simulink model "SITRA_S5_Physical"  (R2026a)
settings: Solver=daessc  StopTime=S5.stopTime  MaxStep=S5.maxStep  RelTol=1e-6  AbsTol=1e-9
values from neighbouring files (symbols this model uses):
  S5 = default_signals(S5)    [build_SITRA_S5_Physical.m]    (also in run_controllers_on_S5_physical.m = evalin('base', 'S5'); test_SITRA_S5_Physical.m = evalin('base', 'S5'); upgrade_electrical_subsystems.m = [model '/05_Power_Electronics'])
libraries: fl_lib x39, nesl_utility x23, ee_lib x9, simulink x8, slpidlib x1
(part 2 of 2)

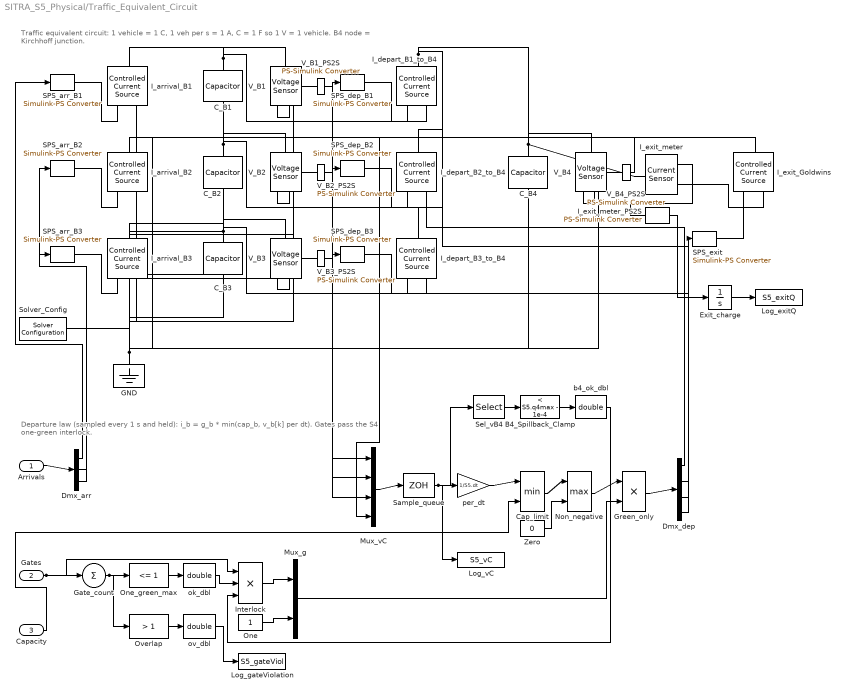
== system SITRA_S5_Physical/Traffic_Equivalent_Circuit ==
  note: Traffic equivalent circuit: 1 vehicle = 1 C, 1 veh per s = 1 A, C = 1 F so 1 V = 1 vehicle. B4 node = Kirchhoff junction.
  note: Departure law (sampled every 1 s and held): i_b = g_b * min(cap_b, v_b[k] per dt). Gates pass the S4 one-green interlock.
  Arrivals : Inport
  Gates : Inport  Port=2
  Capacity : Inport  Port=3
  B4_Spillback_Clamp : simulink/Logic and Bit Operations/Compare To Constant  relop=<  const=S5.q4max - 1e-4  OutDataTypeStr=boolean
  C_B1 : fl_lib/Electrical/Electrical Elements/Capacitor  c=S5.C_queue F  r=1e-6 Ohm  g=0 1/Ohm  i_specify=off  i_priority=None  i=0 A  i_nominal_specify=off  i_nominal_value=1  i_nominal_unit=A  v_specify=off  v_priority=None  v=0 V  v_nominal_specify=off  v_nominal_value=1  v_nominal_unit=V  vc_specify=on  vc_priority=High  vc=S5.vC0(1) V  vc_nominal_specify=off  vc_nominal_value=1  vc_nominal_unit=V
  C_B2 : fl_lib/Electrical/Electrical Elements/Capacitor  c=S5.C_queue F  r=1e-6 Ohm  g=0 1/Ohm  i_specify=off  i_priority=None  i=0 A  i_nominal_specify=off  i_nominal_value=1  i_nominal_unit=A  v_specify=off  v_priority=None  v=0 V  v_nominal_specify=off  v_nominal_value=1  v_nominal_unit=V  vc_specify=on  vc_priority=High  vc=S5.vC0(2) V  vc_nominal_specify=off  vc_nominal_value=1  vc_nominal_unit=V
  C_B3 : fl_lib/Electrical/Electrical Elements/Capacitor  c=S5.C_queue F  r=1e-6 Ohm  g=0 1/Ohm  i_specify=off  i_priority=None  i=0 A  i_nominal_specify=off  i_nominal_value=1  i_nominal_unit=A  v_specify=off  v_priority=None  v=0 V  v_nominal_specify=off  v_nominal_value=1  v_nominal_unit=V  vc_specify=on  vc_priority=High  vc=S5.vC0(3) V  vc_nominal_specify=off  vc_nominal_value=1  vc_nominal_unit=V
  C_B4 : fl_lib/Electrical/Electrical Elements/Capacitor  c=S5.C_queue F  r=1e-6 Ohm  g=0 1/Ohm  i_specify=off  i_priority=None  i=0 A  i_nominal_specify=off  i_nominal_value=1  i_nominal_unit=A  v_specify=off  v_priority=None  v=0 V  v_nominal_specify=off  v_nominal_value=1  v_nominal_unit=V  vc_specify=on  vc_priority=High  vc=S5.vC0(4) V  vc_nominal_specify=off  vc_nominal_value=1  vc_nominal_unit=V
  Cap_limit : MinMax  Inputs=2
  Dmx_arr : Demux  Outputs=3
  Dmx_dep : Demux
  Exit_charge : Integrator
  GND : fl_lib/Electrical/Electrical Elements/Electrical Reference
  Gate_count : Sum  Inputs=+
  Green_only : Product  Inputs=**
  I_arrival_B1 : fl_lib/Electrical/Electrical Sources/Controlled Current Source
  I_arrival_B2 : fl_lib/Electrical/Electrical Sources/Controlled Current Source
  I_arrival_B3 : fl_lib/Electrical/Electrical Sources/Controlled Current Source
  I_depart_B1_to_B4 : fl_lib/Electrical/Electrical Sources/Controlled Current Source
  I_depart_B2_to_B4 : fl_lib/Electrical/Electrical Sources/Controlled Current Source
  I_depart_B3_to_B4 : fl_lib/Electrical/Electrical Sources/Controlled Current Source
  I_exit_Goldwins : fl_lib/Electrical/Electrical Sources/Controlled Current Source
  I_exit_meter : fl_lib/Electrical/Electrical Sensors/Current Sensor
  I_exit_meter_PS2S : nesl_utility/PS-Simulink Converter  PhysicalDomain=network_engine_domain  SubClassName=ps_output  LeftPortType=input  RightPortType=output  PseudoPeriodic=off  Frequencies=[]  VectorFormat=inherit  Unit=A  AffineConversion=off
  Interlock : Product  Inputs=***
  Log_exitQ : ToWorkspace  VariableName=S5_exitQ  SaveFormat=Structure With Time  SampleTime=S5.dt
  Log_gateViolation : ToWorkspace  VariableName=S5_gateViol  SaveFormat=Structure With Time  SampleTime=1
  Log_vC : ToWorkspace  VariableName=S5_vC  SaveFormat=Structure With Time  SampleTime=S5.dt
  Mux_g : Mux  Inputs=2
  Mux_vC : Mux
  Non_negative : MinMax  Function=max  Inputs=2
  One : Constant
  One_green_max : simulink/Logic and Bit Operations/Compare To Constant  relop=<=  const=1  OutDataTypeStr=boolean
  Overlap : simulink/Logic and Bit Operations/Compare To Constant  relop=>  const=1  OutDataTypeStr=boolean
  SPS_arr_B1 : nesl_utility/Simulink-PS Converter  PhysicalDomain=network_engine_domain  SubClassName=ps_input  LeftPortType=input  RightPortType=output  PseudoPeriodic=off  Frequencies=[]  NoiseDistribution=none  NoiseParameters=[]  Unit=A  AffineConversion=off  FilteringAndDerivatives=zero  SimscapeFilterOrder=1  InputFilterTimeConstant=0.001  UdotUserProvided=0
  SPS_arr_B2 : nesl_utility/Simulink-PS Converter  PhysicalDomain=network_engine_domain  SubClassName=ps_input  LeftPortType=input  RightPortType=output  PseudoPeriodic=off  Frequencies=[]  NoiseDistribution=none  NoiseParameters=[]  Unit=A  AffineConversion=off  FilteringAndDerivatives=zero  SimscapeFilterOrder=1  InputFilterTimeConstant=0.001  UdotUserProvided=0
  SPS_arr_B3 : nesl_utility/Simulink-PS Converter  PhysicalDomain=network_engine_domain  SubClassName=ps_input  LeftPortType=input  RightPortType=output  PseudoPeriodic=off  Frequencies=[]  NoiseDistribution=none  NoiseParameters=[]  Unit=A  AffineConversion=off  FilteringAndDerivatives=zero  SimscapeFilterOrder=1  InputFilterTimeConstant=0.001  UdotUserProvided=0
  SPS_dep_B1 : nesl_utility/Simulink-PS Converter  PhysicalDomain=network_engine_domain  SubClassName=ps_input  LeftPortType=input  RightPortType=output  PseudoPeriodic=off  Frequencies=[]  NoiseDistribution=none  NoiseParameters=[]  Unit=A  AffineConversion=off  FilteringAndDerivatives=zero  SimscapeFilterOrder=1  InputFilterTimeConstant=0.001  UdotUserProvided=0
  SPS_dep_B2 : nesl_utility/Simulink-PS Converter  PhysicalDomain=network_engine_domain  SubClassName=ps_input  LeftPortType=input  RightPortType=output  PseudoPeriodic=off  Frequencies=[]  NoiseDistribution=none  NoiseParameters=[]  Unit=A  AffineConversion=off  FilteringAndDerivatives=zero  SimscapeFilterOrder=1  InputFilterTimeConstant=0.001  UdotUserProvided=0
  SPS_dep_B3 : nesl_utility/Simulink-PS Converter  PhysicalDomain=network_engine_domain  SubClassName=ps_input  LeftPortType=input  RightPortType=output  PseudoPeriodic=off  Frequencies=[]  NoiseDistribution=none  NoiseParameters=[]  Unit=A  AffineConversion=off  FilteringAndDerivatives=zero  SimscapeFilterOrder=1  InputFilterTimeConstant=0.001  UdotUserProvided=0
  SPS_exit : nesl_utility/Simulink-PS Converter  PhysicalDomain=network_engine_domain  SubClassName=ps_input  LeftPortType=input  RightPortType=output  PseudoPeriodic=off  Frequencies=[]  NoiseDistribution=none  NoiseParameters=[]  Unit=A  AffineConversion=off  FilteringAndDerivatives=zero  SimscapeFilterOrder=1  InputFilterTimeConstant=0.001  UdotUserProvided=0
  Sample_queue : ZeroOrderHold  SampleTime=S5.dt
  Sel_vB4 : Selector  InputPortWidth=4  IndexOptions=Index vector (dialog)  Indices=4  OutputSizes=1
  Solver_Config : nesl_utility/Solver Configuration  PhysicalDomain=network_engine_domain  SubClassName=solver  LeftPortType=input  RightPortType=generic  Tones=[]  Harmonics=[]  SimulateNoise=off  Profile=off  UseLocalSampling=off  EnableSwitchedLinearOptims=on  FrequencyDomain=off  UseCCode=off  RelTol=0.001  AbsTol=0.001  MinStep=1e-09  ToWorkspace=off  RevertToSquareIcSolve=off  NumHomotopyIterations=100  PhasorMode=off  PhasorModeNumHarmonics=1  ConsistencySolver=NEWTON_XTOL_AFTER_FTOL  CanonicalOrdering=CANONICAL  OptimizeIntermediates=OPTIMIZED  IndexReductionMethod=DerivativeReplacement  DoDC=off  ResidualTolerance=1e-09  ConsistencyTolSource=GLOBAL  ConsistencyAbsTol=0.001  ConsistencyRelTol=0.001  ConsistencyTolFactor=0.001  UseLocalSolver=off  LocalSolverChoice=NE_BACKWARD_EULER_ADVANCER  ResolveIndetEquations=on  FunctionEvalNumThread=1  LocalSolverSampleTime=0.001  DoFixedCost=off  MaxNonlinIter=3  MaxModeIter=2  ComputeImpulses=off  ImpulseIterations=2  LinearAlgebra=auto  LinearAlgebraNumThread=0  EquationFormulation=NE_TIME_EF  DelaysMemoryBudget=1024  AutomaticFiltering=on  FilteringTimeConstant=0.001  PartitionStorageMethod=AS_NEEDED  PartitionMemoryBudget=1024  PartitionMethod=ROBUST  MultibodyUseLocalSolver=off  MultibodyLocalSolverChoice=ODE1  MultibodyLocalSolverSampleTime=0.001
  V_B{1..4} (4 alike) : fl_lib/Electrical/Electrical Sensors/Voltage Sensor
  V_B1_PS2S : nesl_utility/PS-Simulink Converter  PhysicalDomain=network_engine_domain  SubClassName=ps_output  LeftPortType=input  RightPortType=output  PseudoPeriodic=off  Frequencies=[]  VectorFormat=inherit  Unit=V  AffineConversion=off
  V_B2_PS2S : nesl_utility/PS-Simulink Converter  PhysicalDomain=network_engine_domain  SubClassName=ps_output  LeftPortType=input  RightPortType=output  PseudoPeriodic=off  Frequencies=[]  VectorFormat=inherit  Unit=V  AffineConversion=off
  V_B3_PS2S : nesl_utility/PS-Simulink Converter  PhysicalDomain=network_engine_domain  SubClassName=ps_output  LeftPortType=input  RightPortType=output  PseudoPeriodic=off  Frequencies=[]  VectorFormat=inherit  Unit=V  AffineConversion=off
  V_B4_PS2S : nesl_utility/PS-Simulink Converter  PhysicalDomain=network_engine_domain  SubClassName=ps_output  LeftPortType=input  RightPortType=output  PseudoPeriodic=off  Frequencies=[]  VectorFormat=inherit  Unit=V  AffineConversion=off
  Zero : Constant  Value=0
  b4_ok_dbl : DataTypeConversion  OutDataTypeStr=double  SaturateOnIntegerOverflow=off  RndMeth=Floor
  ok_dbl : DataTypeConversion  OutDataTypeStr=double  SaturateOnIntegerOverflow=off  RndMeth=Floor
  ov_dbl : DataTypeConversion  OutDataTypeStr=double  SaturateOnIntegerOverflow=off  RndMeth=Floor
  per_dt : Gain  Gain=1/S5.dt
  wires:
  Arrivals/1 -> Dmx_arr/1
  Dmx_arr/1 -> SPS_arr_B1/1
  Dmx_arr/2 -> SPS_arr_B2/1
  Dmx_arr/3 -> SPS_arr_B3/1
  Gates/1 -> Gate_count/1, Interlock/1
  Gate_count/1 -> One_green_max/1, Overlap/1
  One_green_max/1 -> ok_dbl/1
  ok_dbl/1 -> Interlock/2
  Interlock/1 -> Mux_g/1
  One/1 -> Mux_g/2
  Overlap/1 -> ov_dbl/1
  ov_dbl/1 -> Log_gateViolation/1
  V_B1_PS2S/1 -> Mux_vC/1
  V_B2_PS2S/1 -> Mux_vC/2
  V_B3_PS2S/1 -> Mux_vC/3
  V_B4_PS2S/1 -> Mux_vC/4
  Mux_vC/1 -> Sample_queue/1
  Sample_queue/1 -> Sel_vB4/1, per_dt/1, Log_vC/1
  Sel_vB4/1 -> B4_Spillback_Clamp/1
  B4_Spillback_Clamp/1 -> b4_ok_dbl/1
  b4_ok_dbl/1 -> Interlock/3
  per_dt/1 -> Cap_limit/1
  Capacity/1 -> Cap_limit/2
  Cap_limit/1 -> Non_negative/1
  Zero/1 -> Non_negative/2
  Non_negative/1 -> Green_only/1
  Mux_g/1 -> Green_only/2
  Green_only/1 -> Dmx_dep/1
  Dmx_dep/1 -> SPS_dep_B1/1
  Dmx_dep/2 -> SPS_dep_B2/1
  Dmx_dep/3 -> SPS_dep_B3/1
  Dmx_dep/4 -> SPS_exit/1
  I_exit_meter_PS2S/1 -> Exit_charge/1
  Exit_charge/1 -> Log_exitQ/1
  connections:
  Solver_Config/RConn1 -- I_arrival_B1/RConn2 -- C_B1/RConn1 -- V_B1/RConn2 -- I_arrival_B2/RConn2 -- C_B2/RConn1 -- V_B2/RConn2 -- I_arrival_B3/RConn2 -- C_B3/RConn1 -- V_B3/RConn2 -- C_B4/RConn1 -- V_B4/RConn2 -- GND/LConn1 -- I_exit_Goldwins/LConn1
  SPS_arr_B1/RConn1 -- I_arrival_B1/RConn1
  V_B1/RConn1 -- V_B1_PS2S/LConn1
  SPS_dep_B1/RConn1 -- I_depart_B1_to_B4/RConn1
  I_arrival_B1/LConn1 -- V_B1/LConn1 -- C_B1/LConn1 -- I_depart_B1_to_B4/RConn2
  SPS_arr_B2/RConn1 -- I_arrival_B2/RConn1
  V_B2/RConn1 -- V_B2_PS2S/LConn1
  SPS_dep_B2/RConn1 -- I_depart_B2_to_B4/RConn1
  I_arrival_B2/LConn1 -- V_B2/LConn1 -- C_B2/LConn1 -- I_depart_B2_to_B4/RConn2
  I_depart_B2_to_B4/LConn1 -- I_depart_B3_to_B4/LConn1 -- I_depart_B1_to_B4/LConn1 -- V_B4/LConn1 -- C_B4/LConn1 -- I_exit_meter/LConn1
  SPS_arr_B3/RConn1 -- I_arrival_B3/RConn1
  V_B3/RConn1 -- V_B3_PS2S/LConn1
  SPS_dep_B3/RConn1 -- I_depart_B3_to_B4/RConn1
  I_arrival_B3/LConn1 -- V_B3/LConn1 -- C_B3/LConn1 -- I_depart_B3_to_B4/RConn2
  V_B4/RConn1 -- V_B4_PS2S/LConn1
  I_exit_meter/RConn1 -- I_exit_meter_PS2S/LConn1
  SPS_exit/RConn1 -- I_exit_Goldwins/RConn1
  I_exit_meter/RConn2 -- I_exit_Goldwins/RConn2
